simulink model "demoSemisubDPsystem"  (R2024a)
settings: Solver=ode4  StartTime=0.0  StopTime=1000  FixedStep=0.05  RelTol=1e-3  EnableMultiTasking=on
undefined symbols (not defined in the file): D, slcm
libraries: mssSimulink x4, simulink_extras x2
settings Model: Creator=Thor  LastModifiedBy=thor
settings SolverCC: AlgebraicLoopSolver=TrustRegion  AutoInsertRateTranBlk=on
settings DataIOCC: LimitDataPoints=on  SaveFormat=Array  SignalLoggingSaveFormat=ModelDataLogs  ReturnWorkspaceOutputs=off  SignalLoggingName=sigsOut
settings OptimizationCC: ExpressionDepthLimit=2147483647  InitFltsAndDblsToZero=on  LifeSpan=inf
settings DebuggingCC: SaveWithParameterizedLinksMsg=none  UnderspecifiedInitializationDetection=Classic  MergeDetectMultiDrivingBlocksExec=none  SignalResolutionControl=TryResolveAllWithWarning  MultiTaskDSMMsg=warning  MultiTaskCondExecSysMsg=none  FcnCallInpInsideContextMsg=warning  UnconnectedInputMsg=warning  UnconnectedOutputMsg=warning  UnconnectedLineMsg=warning  StateNameClashWarn=warning  SFUnexpectedBacktrackingDiag=warning  SFNoUnconditionalDefaultTransitionDiag=warning  SFExecutionAtInitializationDiag=none  ArithmeticOperatorsInVariantConditions=warning
settings HardwareCC: ProdBitPerPointer=32  ProdBitPerSizeT=32  ProdBitPerPtrDiffT=32  ProdLargestAtomicFloat=None  ProdIntDivRoundTo=Undefined  ProdEndianess=Unspecified  ProdWordSize=32  ProdHWDeviceType=32-bit Generic  TargetUnknown=on
settings ModelReferenceCC: EnableRefExpFcnMdlSchedulingChecks=on  PropagateSignalLabelsOutOfModel=off
settings SFSimCC: SimUseLocalCustomCode=off  CustomCodeUndefinedFunction=UseInterfaceOnly
settings RTWCC: RTWUseLocalCustomCode=off  GPUComputeCapability=3.5  DLArmComputeVersion=19.05
settings CodeAppCC: StateflowObjectComments=on
settings GRTTargetCC: TargetFcnLib=ansi_tfl_tmw.mat  TargetLangStandard=C89/C90 (ANSI)  ModelReferenceCompliant=off  CombineOutputUpdateFcns=off  MatFileLogging=off  GRTInterface=on
settings ConfigComp: CovMetricSettings=dw  CovSaveCumulativeToWorkspaceVar=on  CovSaveSingleToWorkspaceVar=on  CovExternalEMLEnable=off

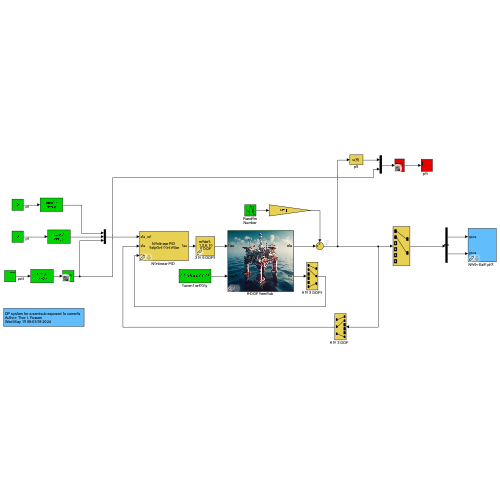
[thumbnail: Simulink's stored preview of the top-level diagram]
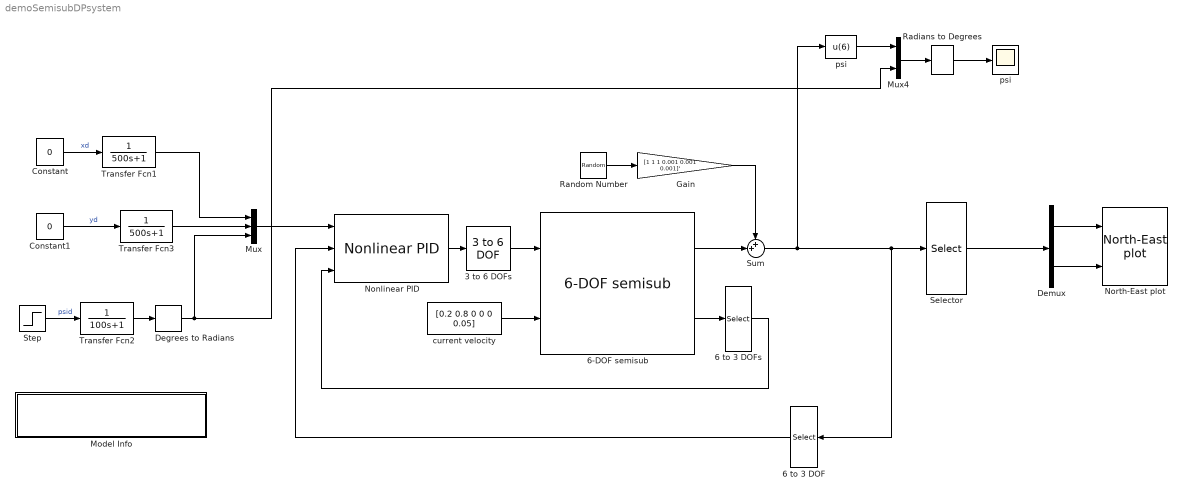
== system demoSemisubDPsystem ==
  3 to 6 DOFs : mssSimulink/Modelling/Kinetics /Support/3 to 6 DOF  SystemSampleTime=-1  VariantActivationTime=update diagram  AllowFlexibleInterface=on  Latency=0  AutoFrameSizeCalculation=off
  "6 to 3 DOF  " : Selector  InputPortWidth=6  IndexOptions=Index vector (dialog)  Indices=[1 2 6]  OutputSizes=1
  6 to 3 DOFs : Selector  InputPortWidth=6  IndexOptions=Index vector (dialog)  Indices=[1 2 6]  OutputSizes=1
  "6-DOF semisub " : mssSimulink/Marine craft models/6-DOF semisub  D=D  G=G  MA=MA  MRB=MRB
  Constant : Constant  Value=0
  Constant1 : Constant  Value=0
  Degrees to Radians : simulink_extras/Transformations/Degrees to Radians
  Demux : Demux  Outputs=2
      settings: DisplayOption=none
  Gain : Gain  Gain=[1 1 1 0.001 0.001 0.001]'
  Model Info : Subsystem  LoadFcn=slcm LoadBlock;  InitFcn=slcm('UpdateAllCMBlocksInThisModelInit')  mask(CMBlock){InitialSaveTempField=, InitialBlockCM=None, BlockCM=None, Frame=on, SaveTempField=, DisplayStringWithTags=|, MaskDisplayString=DP system for a semisub exposed to currents\nAuthor: Thor I. Fossen\nWed May 15 09:03:58 2024, HorizontalTextAlignment=Left, LeftAlignmentValue=0.02, SourceBlockDiagram=demorig, TagMaxNumber=20, CMTag1=, CMTag2=, CMTag3=, CMTag4=, CMTag5=, CMTag6=, CMTag7=, CMTag8=, CMTag9=, CMTag10=, CMTag11=, CMTag12=, CMTag13=, CMTag14=, CMTag15=, CMTag16=, CMTag17=, CMTag18=, CMTag19=, CMTag20=}
      mask DisplayStringWithTags=|
      | DP system for a semisub exposed to currents
      | Author: Thor I. Fossen
      | %<LastModificationDate>
      mask help: This block allows revision control information to be displayed within the model.
      settings: CopyFcn=slcm CopyBlock;  DeleteFcn=slcm Cancel;  PostSaveFcn=slcm('UpdateAllCMBlocksInThisModel')  NameChangeFcn=slcm Rename;  OpenFcn=slcm
      mask Display: text(str2num(LeftAlignmentValue), 0.5, MaskDisplayString, 'HorizontalAlignment', HorizontalTextAlignment)
  Mux : Mux  Inputs=3
  Mux4 : Mux  Inputs=2
  "Nonlinear PID " : mssSimulink/Control/DP/Nonlinear PID  Kp=diag([0.044e10 0.0069e10 6.9241e10])*0.1*0.1  Kd=diag([0.044e10 0.0069e10 6.9241e10])*2*0.1  Ki=diag([0.044e10 0.0069e10 6.9241e10])*(0.1^3)/10
  "North-East plot  " : mssSimulink/Utilities/Visualization/North-East plot    decimation=100
  Radians to Degrees : simulink_extras/Transformations/Radians to Degrees
  Random Number : RandomNumber  Variance=0.1  SampleTime=0.05
  Selector : Selector  InputPortWidth=6  IndexOptions=Index vector (dialog)  Indices=[1 2]  OutputSizes=1
  Step : Step  Time=500  After=30  SampleTime=0
  Sum : Sum  Inputs=++|
  Transfer Fcn1 : TransferFcn  Denominator=[500 1]
  Transfer Fcn2 : TransferFcn  Denominator=[100 1]
  Transfer Fcn3 : TransferFcn  Denominator=[500 1]
  current velocity : Constant  Value=[0.2 0.8 0 0 0 0.05]
  psi : Fcn  Expr=u(6)
  "psi  " : Scope
  wires:
  Constant/1 -> Transfer Fcn1/1  "xd"
  Step/1 -> Transfer Fcn2/1  "psid"
  Degrees to Radians/1 -> Mux4/2, Mux/3
  Constant1/1 -> Transfer Fcn3/1  "yd"
  Demux/1 -> "North-East plot  "/1
  Demux/2 -> "North-East plot  "/2
  Mux/1 -> "Nonlinear PID "/1
  Transfer Fcn2/1 -> Degrees to Radians/1
  Sum/1 -> Selector/1, "6 to 3 DOF  "/1, psi/1
  Radians to Degrees/1 -> "psi  "/1
  Mux4/1 -> Radians to Degrees/1
  "Nonlinear PID "/1 -> 3 to 6 DOFs/1
  psi/1 -> Mux4/1
  Selector/1 -> Demux/1
  current velocity/1 -> "6-DOF semisub "/2
  3 to 6 DOFs/1 -> "6-DOF semisub "/1
  6 to 3 DOFs/1 -> "Nonlinear PID "/3
  "6 to 3 DOF  "/1 -> "Nonlinear PID "/2
  "6-DOF semisub "/2 -> 6 to 3 DOFs/1
  Transfer Fcn1/1 -> Mux/1
  Transfer Fcn3/1 -> Mux/2
  "6-DOF semisub "/1 -> Sum/2
  Random Number/1 -> Gain/1
  Gain/1 -> Sum/1

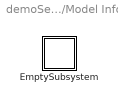
== system demoSemisubDPsystem/Model Info ==
  EmptySubsystem : Subsystem

== system demoSemisubDPsystem/Model Info/EmptySubsystem ==
